simulink library "lib_IC_VSM"  (R2026a)
settings: Solver=VariableStepAuto
undefined symbols (not defined in the file): block_buses, block_DC_buses, block_DC_toM, block_idx, block_toM, buses_lf, DC, dparams, fb, fref, iC, inv2Hv, invL, iR, iTf, omegab, op_intconv_VSM
libraries: sl_discontinuities x1
(part 2 of 3)

== system lib_IC_VSM/intconv_VSM/VI/WOF_q ==
  note: 1) Add Subsystem or Model blocks as valid variant choices.
      | 2) You cannot connect blocks at this level. At simulation, connectivity is automatically
      | determined, based on the active variant and port name matching.
  In1 : Inport
  Active : Subsystem  VariantControl=use_Tf == 1
  Bypass : Subsystem  VariantControl=(default)
  Out1 : Outport

== system lib_IC_VSM/intconv_VSM/DC_ATM_Control/Int_kiw/Active ==
  In1 : Inport
  Impl : Integrator  InitialCondition=op_intconv_VSM.DC_ATM_Control_Int_kiw_Active_Impl
  Out1 : Outport
  wires:
  Impl/1 -> Out1/1
  In1/1 -> Impl/1

== system lib_IC_VSM/intconv_VSM/DC_ATM_Control/Int_kiw/Bypass ==
  In1 : Inport
  Out1 : Outport
  wires:
  In1/1 -> Out1/1

== system lib_IC_VSM/intconv_VSM/DC_ATM_Control/WOF_dc/Active ==
  In1 : Inport
  Impl : Subsystem
  Out1 : Outport
  wires:
  Impl/1(Out1) -> Out1/1
  In1/1 -> Impl/1(In1)

== system lib_IC_VSM/intconv_VSM/DC_ATM_Control/WOF_dc/Bypass ==
  In1 : Inport
  Out1 : Outport
  wires:
  In1/1 -> Out1/1

== system lib_IC_VSM/intconv_VSM/PC/LPF_P/Active ==
  In1 : Inport
  Impl : Subsystem
  Out1 : Outport
  wires:
  Impl/1(P_f) -> Out1/1
  In1/1 -> Impl/1(P)

== system lib_IC_VSM/intconv_VSM/PC/LPF_P/Bypass ==
  In1 : Inport
  Out1 : Outport
  wires:
  In1/1 -> Out1/1

== system lib_IC_VSM/intconv_VSM/PC/LPF_Q/Active ==
  In1 : Inport
  Impl : Subsystem
  Out1 : Outport
  wires:
  Impl/1(Q_f) -> Out1/1
  In1/1 -> Impl/1(Q)

== system lib_IC_VSM/intconv_VSM/PC/LPF_Q/Bypass ==
  In1 : Inport
  Out1 : Outport
  wires:
  In1/1 -> Out1/1

== system lib_IC_VSM/intconv_VSM/PC/Swing/Active ==
  Psp : Inport
  P_f : Inport  Port=2
  omegaref : Inport  Port=3
  Gain_Dv : Gain  Gain=Dv
  Gain_inv2Hv : Gain  Gain=inv2Hv
  Gain_invRv : Gain  Gain=1./Rv
  One_w : Constant  Value=ones(1, length(block_buses))  VectorParams1D=off
  Sum_acc : Sum  Inputs=+---
  Sum_dw_1 : Sum  Inputs=+-
  Sum_dw_ref : Sum  Inputs=+-
  omega_i : Integrator  InitialCondition=op_intconv_VSM.PC_omega_i
  y : Outport
  wires:
  Psp/1 -> Sum_acc/1
  P_f/1 -> Sum_acc/2
  omega_i/1 -> Sum_dw_ref/1, Sum_dw_1/1, y/1
  omegaref/1 -> Sum_dw_ref/2
  Sum_dw_ref/1 -> Gain_invRv/1
  Gain_invRv/1 -> Sum_acc/3
  One_w/1 -> Sum_dw_1/2
  Sum_dw_1/1 -> Gain_Dv/1
  Gain_Dv/1 -> Sum_acc/4
  Sum_acc/1 -> Gain_inv2Hv/1
  Gain_inv2Hv/1 -> omega_i/1

== system lib_IC_VSM/intconv_VSM/PC/Swing/Droop ==
  Psp : Inport
  P_f : Inport  Port=2
  omegaref : Inport  Port=3
  Gain_Rv : Gain  Gain=Rv
  Sum_P : Sum  Inputs=+-
  Sum_w : Sum
  y : Outport
  wires:
  Psp/1 -> Sum_P/1
  P_f/1 -> Sum_P/2
  Sum_P/1 -> Gain_Rv/1
  Gain_Rv/1 -> Sum_w/1
  omegaref/1 -> Sum_w/2
  Sum_w/1 -> y/1

== system lib_IC_VSM/intconv_VSM/VCC/dynamic/PIid ==
  ref : Inport
  y : Inport  Port=2
  Gain : Gain  Gain=Bint
  Gain1 : Gain  Gain=1./Tint
  Gain2 : Gain  Gain=Kint
  I : Integrator  InitialCondition=op_intconv_VSM.VCC_dynamic_PIid_I
  Sum : Sum  Inputs=++|
  Sum1 : Sum  Inputs=|+-
  Sum6 : Sum  Inputs=|+-
  Out1 : Outport
  wires:
  y/1 -> Sum1/2, Sum6/2
  ref/1 -> Gain/1, Sum6/1
  Gain/1 -> Sum1/1
  Sum/1 -> Gain2/1
  Sum1/1 -> Sum/1
  Sum6/1 -> Gain1/1
  Gain1/1 -> I/1
  I/1 -> Sum/2
  Gain2/1 -> Out1/1

== system lib_IC_VSM/intconv_VSM/VCC/dynamic/PIiq ==
  ref : Inport
  y : Inport  Port=2
  Gain : Gain  Gain=Bint
  Gain1 : Gain  Gain=1./Tint
  Gain2 : Gain  Gain=Kint
  I : Integrator  InitialCondition=op_intconv_VSM.VCC_dynamic_PIiq_I
  Sum : Sum  Inputs=++|
  Sum1 : Sum  Inputs=|+-
  Sum6 : Sum  Inputs=|+-
  Out1 : Outport
  wires:
  Gain2/1 -> Out1/1
  I/1 -> Sum/2
  Gain1/1 -> I/1
  Sum6/1 -> Gain1/1
  Sum1/1 -> Sum/1
  Sum/1 -> Gain2/1
  Gain/1 -> Sum1/1
  ref/1 -> Sum6/1, Gain/1
  y/1 -> Sum6/2, Sum1/2

== system lib_IC_VSM/intconv_VSM/VCC/dynamic/PIvd ==
  ref : Inport
  y : Inport  Port=2
  Gain : Gain  Gain=Bext
  Gain1 : Gain  Gain=1./Text
  Gain2 : Gain  Gain=Kext
  Integrator : Integrator  InitialCondition=op_intconv_VSM.VCC_dynamic_PIvd_Integrator
  Sum : Sum  Inputs=++|
  Sum1 : Sum  Inputs=|+-
  Sum6 : Sum  Inputs=|+-
  Out1 : Outport
  wires:
  y/1 -> Sum1/2, Sum6/2
  ref/1 -> Gain/1, Sum6/1
  Gain/1 -> Sum1/1
  Sum/1 -> Gain2/1
  Sum1/1 -> Sum/1
  Sum6/1 -> Gain1/1
  Gain1/1 -> Integrator/1
  Integrator/1 -> Sum/2
  Gain2/1 -> Out1/1

== system lib_IC_VSM/intconv_VSM/VCC/dynamic/PIvq ==
  ref : Inport
  y : Inport  Port=2
  Gain : Gain  Gain=Bext
  Gain1 : Gain  Gain=1./Text
  Gain2 : Gain  Gain=Kext
  Integrator : Integrator  InitialCondition=op_intconv_VSM.VCC_dynamic_PIvq_Integrator
  Sum : Sum  Inputs=++|
  Sum1 : Sum  Inputs=|+-
  Sum6 : Sum  Inputs=|+-
  Out1 : Outport
  wires:
  Gain2/1 -> Out1/1
  Integrator/1 -> Sum/2
  Gain1/1 -> Integrator/1
  Sum6/1 -> Gain1/1
  Sum1/1 -> Sum/1
  Sum/1 -> Gain2/1
  Gain/1 -> Sum1/1
  ref/1 -> Sum6/1, Gain/1
  y/1 -> Sum6/2, Sum1/2

== system lib_IC_VSM/intconv_VSM/VCC/dynamic/RC ==
  note: 1) Add Subsystem or Model blocks as valid variant choices.
      | 2) You cannot connect blocks at this level. At simulation, connectivity is automatically
      | determined, based on the active variant and port name matching.
  i_d_in : Inport
  i_d_out : Inport  Port=2
  i_q_in : Inport  Port=3
  i_q_out : Inport  Port=4
  omega : Inport  Port=5
  dynamic : Subsystem  VariantControl=rc_mode == 1  mask{v_d_0=1}
      mask prompts: v_d_0 "Initial condition for v_d"
  static : Subsystem  VariantControl=rc_mode == 2
  static omega : Subsystem  VariantControl=(default)
  vd : Outport
  vq : Outport  Port=2

== system lib_IC_VSM/intconv_VSM/VCC/dynamic/RL ==
  note: 1) Add Subsystem or Model blocks as valid variant choices.
      | 2) You cannot connect blocks at this level. At simulation, connectivity is automatically
      | determined, based on the active variant and port name matching.
  v_in_d : Inport
  v_out_d : Inport  Port=2
  v_in_q : Inport  Port=3
  v_out_q : Inport  Port=4
  dynamic : Subsystem  VariantControl=rl_mode == 1
      settings: PortSchema="{\"entries\":[{\"content\":{\"sides\":[{\"content\":{\"connectorIds\":[\"In1\"]},\"type\":\"ConnectorPlacement.EquallySpacedRectSide\",\"uuid\":\"63966e24-f9e7-4b2d-b456-7f4ea5e3f230\"},{\"content\":{\"connectorIds\":[\"In2\",\"In3\",\"In4\",\"Out1\",\"Out2\"],\"side\":\"RIGHT\"},\"type\":\"ConnectorPlacement.EquallySpacedRectSide\",\"uuid\":\"ded6ef04-52fd-47df-8e49-cf16b827098d\"},{\"content\":{\"connectorIds\":[],\"side\":\"TOP\"},\"type\":\"ConnectorPlacement.EquallySpacedRectSide\",\"uuid\":\"f940a985-fa23-4968-ad44-1d76d0e20c6a\"}]},\"type\":\"ConnectorPlacement.EquallySpacedConnector\",\"uuid\":\"20f61d3c-9af2-4982-98ea-af4910e61c9c\"}],\"packageUris\":[\"http://schema.mathworks.com/mf0/Connector/R2020b\"],\"version\":\"1.0\"}"
  static : Subsystem  VariantControl=rl_mode == 2
  static_omega : Subsystem  VariantControl=(default)
  id : Outport
  iq : Outport  Port=2

== system lib_IC_VSM/intconv_VSM/VCC/dynamic_VC/RC ==
  note: 1) Add Subsystem or Model blocks as valid variant choices.
      | 2) You cannot connect blocks at this level. At simulation, connectivity is automatically
      | determined, based on the active variant and port name matching.
  i_d_in : Inport
  i_d_out : Inport  Port=2
  i_q_in : Inport  Port=3
  i_q_out : Inport  Port=4
  omega : Inport  Port=5
  dynamic : Subsystem  VariantControl=rc_mode == 1  mask{v_d_0=1}
      mask prompts: v_d_0 "Initial condition for v_d"
  static : Subsystem  VariantControl=rc_mode == 2
  static omega : Subsystem  VariantControl=(default)
  v_d : Outport
  v_q : Outport  Port=2

== system lib_IC_VSM/intconv_VSM/VCC/dynamic_VC/Subsystem ==
  ref : Inport
  y : Inport  Port=2
  Gain : Gain  Gain=Bext
  Gain1 : Gain  Gain=1./Text
  Gain2 : Gain  Gain=Kext
  Integrator : Integrator  InitialCondition=op_intconv_VSM.VCC_dynamic_VC_Subsystem_Integrator
  Sum : Sum  Inputs=++|
  Sum1 : Sum  Inputs=|+-
  Sum6 : Sum  Inputs=|+-
  Out1 : Outport
  wires:
  y/1 -> Sum1/2, Sum6/2
  ref/1 -> Gain/1, Sum6/1
  Gain/1 -> Sum1/1
  Sum/1 -> Gain2/1
  Sum1/1 -> Sum/1
  Sum6/1 -> Gain1/1
  Gain1/1 -> Integrator/1
  Integrator/1 -> Sum/2
  Gain2/1 -> Out1/1

== system lib_IC_VSM/intconv_VSM/VCC/dynamic_VC/Subsystem1 ==
  ref : Inport
  y : Inport  Port=2
  Gain : Gain  Gain=Bext
  Gain1 : Gain  Gain=1./Text
  Gain2 : Gain  Gain=Kext
  Integrator : Integrator  InitialCondition=op_intconv_VSM.VCC_dynamic_VC_Subsystem1_Integrator
  Sum : Sum  Inputs=++|
  Sum1 : Sum  Inputs=|+-
  Sum6 : Sum  Inputs=|+-
  Out1 : Outport
  wires:
  Gain2/1 -> Out1/1
  Integrator/1 -> Sum/2
  Gain1/1 -> Integrator/1
  Sum6/1 -> Gain1/1
  Sum1/1 -> Sum/1
  Sum/1 -> Gain2/1
  Gain/1 -> Sum1/1
  ref/1 -> Sum6/1, Gain/1
  y/1 -> Sum6/2, Sum1/2

== system lib_IC_VSM/intconv_VSM/VCC/dynamic_limiting/PIid ==
  ref : Inport
  y : Inport  Port=2
  Gain : Gain  Gain=Bint
  Gain1 : Gain  Gain=1./Tint
  Gain2 : Gain  Gain=Kint
  I : Integrator  InitialCondition=op_intconv_VSM.VCC_dynamic_limiting_PIid_I
  Sum : Sum  Inputs=++|
  Sum1 : Sum  Inputs=|+-
  Sum6 : Sum  Inputs=|+-
  Out1 : Outport
  wires:
  y/1 -> Sum1/2, Sum6/2
  ref/1 -> Gain/1, Sum6/1
  Gain/1 -> Sum1/1
  Sum/1 -> Gain2/1
  Sum1/1 -> Sum/1
  Sum6/1 -> Gain1/1
  Gain1/1 -> I/1
  I/1 -> Sum/2
  Gain2/1 -> Out1/1

== system lib_IC_VSM/intconv_VSM/VCC/dynamic_limiting/PIiq ==
  ref : Inport
  y : Inport  Port=2
  Gain : Gain  Gain=Bint
  Gain1 : Gain  Gain=1./Tint
  Gain2 : Gain  Gain=Kint
  I : Integrator  InitialCondition=op_intconv_VSM.VCC_dynamic_limiting_PIiq_I
  Sum : Sum  Inputs=++|
  Sum1 : Sum  Inputs=|+-
  Sum6 : Sum  Inputs=|+-
  Out1 : Outport
  wires:
  Gain2/1 -> Out1/1
  I/1 -> Sum/2
  Gain1/1 -> I/1
  Sum6/1 -> Gain1/1
  Sum1/1 -> Sum/1
  Sum/1 -> Gain2/1
  Gain/1 -> Sum1/1
  ref/1 -> Sum6/1, Gain/1
  y/1 -> Sum6/2, Sum1/2

== system lib_IC_VSM/intconv_VSM/VCC/dynamic_limiting/PIvd ==
  ref : Inport
  y : Inport  Port=2
  anti_windup : Inport  Port=3
  Gain : Gain  Gain=Bext
  Gain1 : Gain  Gain=1./Text
  Gain2 : Gain  Gain=Kext
  I : Integrator  InitialCondition=op_intconv_VSM.VCC_dynamic_limiting_PIvd_I
  Product : Product
  Scope : Scope
      settings: ActiveDisplayYMinimum=-5E-5  ActiveDisplayYMaximum=0.00079  DataLoggingVariableName=ScopeData5
  Scope1 : Scope
      settings: ActiveDisplayYMinimum=-0.29497  ActiveDisplayYMaximum=2.2504  DataLoggingVariableName=ScopeData7
  Sum : Sum  Inputs=++|
  Sum1 : Sum  Inputs=|+-
  Sum6 : Sum  Inputs=|+-
  Out1 : Outport
  wires:
  y/1 -> Sum1/2, Sum6/2
  ref/1 -> Gain/1, Sum6/1
  Gain/1 -> Sum1/1
  Sum/1 -> Gain2/1
  Sum1/1 -> Sum/1
  Sum6/1 -> Scope1/1, Gain1/1
  Product/1 -> I/1
  I/1 -> Scope/1, Sum/2
  Gain2/1 -> Out1/1
  Gain1/1 -> Product/1
  anti_windup/1 -> Product/2

== system lib_IC_VSM/intconv_VSM/VCC/dynamic_limiting/PIvq ==
  ref : Inport
  y : Inport  Port=2
  anti_windup : Inport  Port=3
  Gain : Gain  Gain=Bext
  Gain1 : Gain  Gain=1./Text
  Gain2 : Gain  Gain=Kext
  I : Integrator  InitialCondition=op_intconv_VSM.VCC_dynamic_limiting_PIvq_I
  Product : Product
  Sum : Sum  Inputs=++|
  Sum1 : Sum  Inputs=|+-
  Sum6 : Sum  Inputs=|+-
  Out1 : Outport
  wires:
  Gain2/1 -> Out1/1
  I/1 -> Sum/2
  Product/1 -> I/1
  Sum6/1 -> Gain1/1
  Sum1/1 -> Sum/1
  Sum/1 -> Gain2/1
  Gain/1 -> Sum1/1
  ref/1 -> Sum6/1, Gain/1
  y/1 -> Sum6/2, Sum1/2
  Gain1/1 -> Product/1
  anti_windup/1 -> Product/2

== system lib_IC_VSM/intconv_VSM/VCC/dynamic_limiting/RC ==
  note: 1) Add Subsystem or Model blocks as valid variant choices.
      | 2) You cannot connect blocks at this level. At simulation, connectivity is automatically
      | determined, based on the active variant and port name matching.
  i_d_in : Inport
  i_d_out : Inport  Port=2
  i_q_in : Inport  Port=3
  i_q_out : Inport  Port=4
  omega : Inport  Port=5
  dynamic : Subsystem  VariantControl=rc_mode == 1
  static : Subsystem  VariantControl=rc_mode == 2
  static omega : Subsystem  VariantControl=(default)
  vd : Outport
  vq : Outport  Port=2

== system lib_IC_VSM/intconv_VSM/VCC/dynamic_limiting/RL ==
  note: 1) Add Subsystem or Model blocks as valid variant choices.
      | 2) You cannot connect blocks at this level. At simulation, connectivity is automatically
      | determined, based on the active variant and port name matching.
  v_in_d : Inport
  v_out_d : Inport  Port=2
  v_in_q : Inport  Port=3
  v_out_q : Inport  Port=4
  omega : Inport  Port=5
  dynamic : Subsystem  VariantControl=rl_mode == 1
      settings: PortSchema="{\"entries\":[{\"content\":{\"sides\":[{\"content\":{\"connectorIds\":[\"In1\"]},\"type\":\"ConnectorPlacement.EquallySpacedRectSide\",\"uuid\":\"63966e24-f9e7-4b2d-b456-7f4ea5e3f230\"},{\"content\":{\"connectorIds\":[\"In2\",\"In3\",\"In4\",\"In5\",\"Out1\",\"Out2\"],\"side\":\"RIGHT\"},\"type\":\"ConnectorPlacement.EquallySpacedRectSide\",\"uuid\":\"ded6ef04-52fd-47df-8e49-cf16b827098d\"},{\"content\":{\"side\":\"TOP\"},\"type\":\"ConnectorPlacement.EquallySpacedRectSide\",\"uuid\":\"f940a985-fa23-4968-ad44-1d76d0e20c6a\"}]},\"type\":\"ConnectorPlacement.EquallySpacedConnector\",\"uuid\":\"20f61d3c-9af2-4982-98ea-af4910e61c9c\"}],\"packageUris\":[\"http://schema.mathworks.com/mf0/Connector/R2020b\"],\"version\":\"1.0\"}"
  static : Subsystem  VariantControl=rl_mode == 2
  static_omega : Subsystem  VariantControl=(default)
  id : Outport
  iq : Outport  Port=2

== system lib_IC_VSM/intconv_VSM/VCC/dynamic_limiting/VI ==
  id : Inport
  iq : Inport  Port=2
  Gain : Gain  Gain=L
  Gain1 : Gain  Gain=R
  Gain2 : Gain  Gain=L
  Gain3 : Gain  Gain=R
  LPF_omega : Subsystem
  LPF_omega1 : Subsystem
  Sum : Sum  Inputs=-+|
  Sum1 : Sum  Inputs=|--
  WOF_d : Subsystem  Variant=on
  WOF_q : Subsystem  Variant=on
  vd : Outport
  vq : Outport  Port=2
  wires:
  WOF_q/1(Out1) -> Gain/1, Gain3/1
  iq/1 -> WOF_q/1(In1)
  WOF_d/1(Out1) -> Gain1/1, Gain2/1
  id/1 -> WOF_d/1(In1)
  Sum1/1 -> LPF_omega1/1(in)
  Sum/1 -> LPF_omega/1(in)
  Gain3/1 -> Sum1/2
  Gain1/1 -> Sum/1
  Gain2/1 -> Sum1/1
  Gain/1 -> Sum/2
  LPF_omega/1(out) -> vd/1
  LPF_omega1/1(out) -> vq/1

== system lib_IC_VSM/intconv_VSM/VCC/dynamic_limiting_P/PIid ==
  ref : Inport
  y : Inport  Port=2
  Gain : Gain  Gain=Bint
  Gain1 : Gain  Gain=1./Tint
  Gain2 : Gain  Gain=Kint
  I : Integrator  InitialCondition=op_intconv_VSM.VCC_dynamic_limiting_P_PIid_I
  Sum : Sum  Inputs=++|
  Sum1 : Sum  Inputs=|+-
  Sum6 : Sum  Inputs=|+-
  Out1 : Outport
  wires:
  y/1 -> Sum1/2, Sum6/2
  ref/1 -> Gain/1, Sum6/1
  Gain/1 -> Sum1/1
  Sum/1 -> Gain2/1
  Sum1/1 -> Sum/1
  Sum6/1 -> Gain1/1
  Gain1/1 -> I/1
  I/1 -> Sum/2
  Gain2/1 -> Out1/1

== system lib_IC_VSM/intconv_VSM/VCC/dynamic_limiting_P/PIiq ==
  ref : Inport
  y : Inport  Port=2
  Gain : Gain  Gain=Bint
  Gain1 : Gain  Gain=1./Tint
  Gain2 : Gain  Gain=Kint
  I : Integrator  InitialCondition=op_intconv_VSM.VCC_dynamic_limiting_P_PIiq_I
  Sum : Sum  Inputs=++|
  Sum1 : Sum  Inputs=|+-
  Sum6 : Sum  Inputs=|+-
  Out1 : Outport
  wires:
  Gain2/1 -> Out1/1
  I/1 -> Sum/2
  Gain1/1 -> I/1
  Sum6/1 -> Gain1/1
  Sum1/1 -> Sum/1
  Sum/1 -> Gain2/1
  Gain/1 -> Sum1/1
  ref/1 -> Sum6/1, Gain/1
  y/1 -> Sum6/2, Sum1/2

== system lib_IC_VSM/intconv_VSM/VCC/dynamic_limiting_P/PIvd ==
  ref : Inport
  y : Inport  Port=2
  awp : Inport  Port=3
  Gain : Gain  Gain=Bext
  Gain1 : Gain  Gain=1./Text
  Gain2 : Gain  Gain=Kext
  I : Integrator  InitialCondition=op_intconv_VSM.VCC_dynamic_limiting_P_PIvd_I
  Product : Product
  Sum : Sum  Inputs=++|
  Sum1 : Sum  Inputs=|+-
  Sum6 : Sum  Inputs=|+-
  Out1 : Outport
  wires:
  y/1 -> Sum1/2, Sum6/2
  ref/1 -> Gain/1, Sum6/1
  Gain/1 -> Sum1/1
  Sum/1 -> Gain2/1
  Sum1/1 -> Sum/1
  Sum6/1 -> Gain1/1
  Product/1 -> I/1
  Gain1/1 -> Product/1
  I/1 -> Sum/2
  awp/1 -> Product/2
  Gain2/1 -> Out1/1

== system lib_IC_VSM/intconv_VSM/VCC/dynamic_limiting_P/PIvq ==
  ref : Inport
  y : Inport  Port=2
  awp : Inport  Port=3
  Gain : Gain  Gain=Bext
  Gain1 : Gain  Gain=1./Text
  Gain2 : Gain  Gain=Kext
  I : Integrator  InitialCondition=op_intconv_VSM.VCC_dynamic_limiting_P_PIvq_I
  Product : Product
  Sum : Sum  Inputs=++|
  Sum1 : Sum  Inputs=|+-
  Sum6 : Sum  Inputs=|+-
  Out1 : Outport
  wires:
  I/1 -> Sum/2
  Sum6/1 -> Gain1/1
  Sum1/1 -> Sum/1
  Sum/1 -> Gain2/1
  Gain/1 -> Sum1/1
  ref/1 -> Sum6/1, Gain/1
  y/1 -> Sum6/2, Sum1/2
  Gain2/1 -> Out1/1
  Gain1/1 -> I/1, Product/1
  awp/1 -> Product/2

== system lib_IC_VSM/intconv_VSM/VCC/dynamic_limiting_P/RC ==
  note: 1) Add Subsystem or Model blocks as valid variant choices.
      | 2) You cannot connect blocks at this level. At simulation, connectivity is automatically
      | determined, based on the active variant and port name matching.
  i_d_in : Inport
  i_d_out : Inport  Port=2
  i_q_in : Inport  Port=3
  i_q_out : Inport  Port=4
  omega : Inport  Port=5
  dynamic : Subsystem  VariantControl=rc_mode == 1
  static : Subsystem  VariantControl=rc_mode == 2
  static omega : Subsystem  VariantControl=(default)
  vd : Outport
  vq : Outport  Port=2

== system lib_IC_VSM/intconv_VSM/VCC/dynamic_limiting_P/RL ==
  note: 1) Add Subsystem or Model blocks as valid variant choices.
      | 2) You cannot connect blocks at this level. At simulation, connectivity is automatically
      | determined, based on the active variant and port name matching.
  v_in_d : Inport
  v_out_d : Inport  Port=2
  v_in_q : Inport  Port=3
  v_out_q : Inport  Port=4
  omega : Inport  Port=5
  dynamic : Subsystem  VariantControl=rl_mode == 1
      settings: PortSchema="{\"entries\":[{\"content\":{\"sides\":[{\"content\":{\"connectorIds\":[\"In1\"]},\"type\":\"ConnectorPlacement.EquallySpacedRectSide\",\"uuid\":\"63966e24-f9e7-4b2d-b456-7f4ea5e3f230\"},{\"content\":{\"connectorIds\":[\"In2\",\"In3\",\"In4\",\"In5\",\"Out1\",\"Out2\"],\"side\":\"RIGHT\"},\"type\":\"ConnectorPlacement.EquallySpacedRectSide\",\"uuid\":\"ded6ef04-52fd-47df-8e49-cf16b827098d\"},{\"content\":{\"side\":\"TOP\"},\"type\":\"ConnectorPlacement.EquallySpacedRectSide\",\"uuid\":\"f940a985-fa23-4968-ad44-1d76d0e20c6a\"}]},\"type\":\"ConnectorPlacement.EquallySpacedConnector\",\"uuid\":\"20f61d3c-9af2-4982-98ea-af4910e61c9c\"}],\"packageUris\":[\"http://schema.mathworks.com/mf0/Connector/R2020b\"],\"version\":\"1.0\"}"
  static : Subsystem  VariantControl=rl_mode == 2
  static_omega : Subsystem  VariantControl=(default)
  id : Outport
  iq : Outport  Port=2

== system lib_IC_VSM/intconv_VSM/VCC/dynamic_limiting_P/Subsystem2 ==
  In1 : Inport
  In2 : Inport  Port=2
  imax : Inport  Port=3
  Complex to Magnitude-Angle1 : ComplexToMagnitudeAngle
  Complex to Real-Imag : ComplexToRealImag
  Constant1 : Constant  Value=0
  Magnitude-Angle to Complex : MagnitudeAngleToComplex
  Real-Imag to Complex2 : RealImagToComplex
  Relational Operator : RelationalOperator  Operator===  OutDataTypeStr=boolean  RndMeth=Simplest  InputSameDT=off
  Saturation Dynamic1 : sl_discontinuities/Saturation Dynamic  OutMin=[]  OutMax=[]  OutDataTypeStr=Inherit: Same as second input  OutDataType=fixdt(1, 16)  OutScaling=2^-10  DoSatur=off
  ref : Outport
  Out2 : Outport  Port=2
  awp : Outport  Port=3
  wires:
  Constant1/1 -> Saturation Dynamic1/3
  In1/1 -> Real-Imag to Complex2/1
  Complex to Magnitude-Angle1/2 -> Magnitude-Angle to Complex/2
  In2/1 -> Real-Imag to Complex2/2
  Saturation Dynamic1/1 -> Relational Operator/2, Magnitude-Angle to Complex/1
  Complex to Magnitude-Angle1/1 -> Relational Operator/1, Saturation Dynamic1/2
  imax/1 -> Saturation Dynamic1/1
  Magnitude-Angle to Complex/1 -> Complex to Real-Imag/1
  Real-Imag to Complex2/1 -> Complex to Magnitude-Angle1/1
  Complex to Real-Imag/1 -> ref/1
  Complex to Real-Imag/2 -> Out2/1
  Relational Operator/1 -> awp/1

== system lib_IC_VSM/intconv_VSM/VCC/dynamic_limiting_P/VI ==
  id : Inport
  iq : Inport  Port=2
  Gain : Gain  Gain=L
  Gain1 : Gain  Gain=R
  Gain2 : Gain  Gain=L
  Gain3 : Gain  Gain=R
  LPF_omega : Subsystem
  LPF_omega1 : Subsystem
  Sum : Sum  Inputs=-+|
  Sum1 : Sum  Inputs=|--
  WOF_d : Subsystem  Variant=on
  WOF_q : Subsystem  Variant=on
  vd : Outport
  vq : Outport  Port=2
  wires:
  WOF_q/1(Out1) -> Gain/1, Gain3/1
  iq/1 -> WOF_q/1(In1)
  WOF_d/1(Out1) -> Gain1/1, Gain2/1
  id/1 -> WOF_d/1(In1)
  Sum1/1 -> LPF_omega1/1(in)
  Sum/1 -> LPF_omega/1(in)
  Gain3/1 -> Sum1/2
  Gain1/1 -> Sum/1
  Gain2/1 -> Sum1/1
  Gain/1 -> Sum/2
  LPF_omega/1(out) -> vd/1
  LPF_omega1/1(out) -> vq/1

== system lib_IC_VSM/intconv_VSM/VI/WOF_d/Active ==
  In1 : Inport
  Impl : Subsystem
  Out1 : Outport
  wires:
  Impl/1(Out1) -> Out1/1
  In1/1 -> Impl/1(In1)

== system lib_IC_VSM/intconv_VSM/VI/WOF_d/Bypass ==
  In1 : Inport
  Out1 : Outport
  wires:
  In1/1 -> Out1/1

== system lib_IC_VSM/intconv_VSM/VI/WOF_q/Active ==
  In1 : Inport
  Impl : Subsystem
  Out1 : Outport
  wires:
  Impl/1(Out1) -> Out1/1
  In1/1 -> Impl/1(In1)

== system lib_IC_VSM/intconv_VSM/VI/WOF_q/Bypass ==
  In1 : Inport
  Out1 : Outport
  wires:
  In1/1 -> Out1/1

== system lib_IC_VSM/intconv_VSM/DC_ATM_Control/WOF_dc/Active/Impl ==
  In1 : Inport
  Gain : Gain  Gain=N_dc
  Gain1 : Gain  Gain=10
  I : Integrator  InitialConditionSource=external  InitialCondition=op_intconv_VSM.DC_ATM_Control_WOF_dc_Active_Impl_I
  Sum : Sum  Inputs=+-|
  Sum4 : Sum  Inputs=|+-
  Out1 : Outport
  wires:
  Gain/1 -> I/1
  Sum4/1 -> Gain/1
  In1/1 -> I/2, Sum/1, Sum4/1
  I/1 -> Sum/2, Sum4/2
  Sum/1 -> Gain1/1
  Gain1/1 -> Out1/1

== system lib_IC_VSM/intconv_VSM/PC/LPF_P/Active/Impl ==
  P : Inport
  Gain : Gain  Gain=iTf
  I : Integrator  InitialCondition=op_intconv_VSM.PC_LPF_P_Active_Impl_I
  Sum4 : Sum  Inputs=|+-
  P_f : Outport
  wires:
  I/1 -> Sum4/2, P_f/1
  P/1 -> Sum4/1
  Sum4/1 -> Gain/1
  Gain/1 -> I/1

== system lib_IC_VSM/intconv_VSM/PC/LPF_Q/Active/Impl ==
  Q : Inport
  Gain : Gain  Gain=iTf
  I : Integrator  InitialCondition=op_intconv_VSM.PC_LPF_Q_Active_Impl_I
  Sum4 : Sum  Inputs=|+-
  Q_f : Outport
  wires:
  Sum4/1 -> Gain/1
  I/1 -> Sum4/2, Q_f/1
  Q/1 -> Sum4/1
  Gain/1 -> I/1

== system lib_IC_VSM/intconv_VSM/VCC/dynamic/RC/dynamic ==
  omega : Inport
  i_d_in : Inport  Port=2
  i_d_out : Inport  Port=3
  i_q_in : Inport  Port=4
  i_q_out : Inport  Port=5
  Gain1 : Gain  Gain=iR
  Gain2 : Gain  Gain=iR
  Gain3 : Gain  Gain=C
  Gain4 : Gain  Gain=C
  Gain5 : Gain  Gain=iC.*omegab
  Gain6 : Gain  Gain=iC.*omegab
  Product : Product
  Product1 : Product
  Sum10 : Sum  Inputs=|-++
  Sum11 : Sum  Inputs=-+|
  Sum12 : Sum  Inputs=|+-
  Sum13 : Sum  Inputs=-+-|
  v_d : Integrator  InitialCondition=op_intconv_VSM.VCC_dynamic_RC_dynamic_v_d
  v_q : Integrator  InitialCondition=op_intconv_VSM.VCC_dynamic_RC_dynamic_v_q
  vd : Outport
  vq : Outport  Port=2
  wires:
  Sum10/1 -> Gain6/1
  Gain3/1 -> Product1/1
  v_q/1 -> vq/1, Gain2/1, Gain3/1  "vq"
  Product1/1 -> Sum10/3
  Gain4/1 -> Product/1
  Gain2/1 -> Sum13/3
  Product/1 -> Sum13/1
  Sum11/1 -> Sum10/2
  Gain6/1 -> v_d/1
  omega/1 -> Product/2, Product1/2  "omega"
  Sum13/1 -> Gain5/1
  Gain1/1 -> Sum10/1
  Gain5/1 -> v_q/1
  Sum12/1 -> Sum13/2
  v_d/1 -> Gain4/1, vd/1, Gain1/1  "vd"
  i_d_in/1 -> Sum11/2  "id1"
  i_d_out/1 -> Sum11/1  "id2"
  i_q_in/1 -> Sum12/1  "iq1"
  i_q_out/1 -> Sum12/2  "iq2"

== system lib_IC_VSM/intconv_VSM/VCC/dynamic/RC/static ==
  omega : Inport
  i_d_in : Inport  Port=2
  i_d_out : Inport  Port=3
  i_q_in : Inport  Port=4
  i_q_out : Inport  Port=5
  Constant : Constant  Value=iR.^2
  Constant1 : Constant
  Divide : Product  Inputs=*/
  Gain : Gain  Gain=C
  Gain1 : Gain  Gain=iR
  Gain2 : Gain  Gain=iR
  Product{,1..5} (6 alike) : Product
  Sum : Sum  Inputs=|++
  Sum1 : Sum  Inputs=|-+
  Sum2 : Sum  Inputs=|+-
  Sum3 : Sum  Inputs=|++
  Sum4 : Sum  Inputs=|-+
  vd : Outport
  vq : Outport  Port=2
  wires:
  Product5/1 -> Sum4/2
  Gain2/1 -> Product5/2
  Product4/1 -> Sum4/1
  Product2/1 -> Product3/1, Product4/2
  Product3/1 -> Sum3/2
  Product1/1 -> Sum3/1
  Divide/1 -> Product2/1, Gain1/1, Product5/1
  Gain1/1 -> Product1/2
  Sum2/1 -> Product3/2, Gain2/1  "iq"
  Sum1/1 -> Product4/1, Product1/1  "id"
  Constant1/1 -> Divide/1
  Product/1 -> Sum/2
  Gain/1 -> Product/1, Product/2, Product2/2
  Sum/1 -> Divide/2
  Constant/1 -> Sum/1
  Sum4/1 -> vq/1  "vq"
  Sum3/1 -> vd/1  "vd"
  omega/1 -> Gain/1  "omega"
  i_d_in/1 -> Sum1/2  "id1"
  i_q_in/1 -> Sum1/1  "id2"
  i_d_out/1 -> Sum2/1  "iq1"
  i_q_out/1 -> Sum2/2  "iq2"

== system lib_IC_VSM/intconv_VSM/VCC/dynamic/RC/static omega ==
  i_d_in : Inport
  i_d_out : Inport  Port=2
  i_q_in : Inport  Port=3
  i_q_out : Inport  Port=4
  Gain : Gain  Gain=1./(iR.^2+C.^2)
  Gain2 : Gain  Gain=1./(iR.^2+C.^2)
  Gain3 : Gain  Gain=iR
  Gain4 : Gain  Gain=C
  Gain5 : Gain  Gain=iR
  Gain6 : Gain  Gain=C
  Sum : Sum  Inputs=|++
  Sum1 : Sum  Inputs=|+-
  Sum2 : Sum  Inputs=|+-
  Sum4 : Sum  Inputs=|-+
  vd : Outport
  vq : Outport  Port=2
  wires:
  i_q_in/1 -> Sum2/1  "iq1"
  Sum1/1 -> Gain/1  "id"
  Sum2/1 -> Gain2/1  "iq"
  i_q_out/1 -> Sum2/2  "iq2"
  i_d_in/1 -> Sum1/1  "id"
  i_d_out/1 -> Sum1/2
  Gain/1 -> Gain4/1, Gain3/1
  Gain2/1 -> Gain6/1, Gain5/1
  Gain3/1 -> Sum/1
  Gain6/1 -> Sum/2
  Gain4/1 -> Sum4/1
  Gain5/1 -> Sum4/2
  Sum4/1 -> vq/1
  Sum/1 -> vd/1

== system lib_IC_VSM/intconv_VSM/VCC/dynamic/RL/dynamic ==
  v_in_d : Inport
  v_out_d : Inport  Port=2
  v_in_q : Inport  Port=3
  v_out_q : Inport  Port=4
  Gain1 : Gain  Gain=L
  Gain2 : Gain  Gain=R
  Gain3 : Gain  Gain=R
  Gain4 : Gain  Gain=L
  Gain5 : Gain  Gain=invL.*omegab
  Gain7 : Gain  Gain=invL.*omegab
  Product : Product
  Product1 : Product
  Sum4 : Sum  Inputs=+-|
  Sum5 : Sum  Inputs=|-+
  Sum6 : Sum  Inputs=|++
  Sum7 : Sum  Inputs=-+|
  Sum8 : Sum  Inputs=|+-
  Sum9 : Sum  Inputs=-+|
  i_d : Integrator  InitialCondition=op_intconv_VSM.VCC_dynamic_RL_dynamic_i_d
  i_q : Integrator  InitialCondition=op_intconv_VSM.VCC_dynamic_RL_dynamic_i_q
  id : Outport
  iq : Outport  Port=2
  wires:
  v_out_q/1 -> Sum9/1  "v_out_q"
  v_out_d/1 -> Sum7/1  "v_out_d"
  Sum9/1 -> Sum8/1
  Gain1/1 -> Product1/2
  i_q/1 -> iq/1, Gain4/1, Gain3/1  "iq"
  Gain7/1 -> i_q/1
  Sum5/1 -> Sum9/2
  Gain3/1 -> Sum5/1
  Sum7/1 -> Sum6/1
  Gain4/1 -> Product/1
  Product1/1 -> Sum8/2
  Sum4/1 -> Sum7/2
  Sum8/1 -> Gain7/1
  Product/1 -> Sum6/2
  Gain5/1 -> i_d/1
  [omega_ref] -> Product/2, Product1/1  "omega"
  Sum6/1 -> Gain5/1
  i_d/1 -> id/1, Gain1/1, Gain2/1  "id"
  Gain2/1 -> Sum4/2
  v_in_d/1 -> Sum4/1  "v_in_d"
  v_in_q/1 -> Sum5/2  "v_in_q"

== system lib_IC_VSM/intconv_VSM/VCC/dynamic/RL/static ==
  v_in_d : Inport
  v_out_d : Inport  Port=2
  v_in_q : Inport  Port=3
  v_out_q : Inport  Port=4
  Constant : Constant  Value=R.^2
  Constant1 : Constant
  Divide : Product  Inputs=*/
  Gain : Gain  Gain=L
  Gain1 : Gain  Gain=R
  Gain2 : Gain  Gain=R
  Product{,1..5} (6 alike) : Product
  Sum : Sum  Inputs=|++
  Sum1 : Sum  Inputs=|+-
  Sum2 : Sum  Inputs=|+-
  Sum3 : Sum  Inputs=|++
  Sum4 : Sum  Inputs=|-+
  id : Outport
  iq : Outport  Port=2
  wires:
  [omega_ref] -> Gain/1  "omega"
  v_in_d/1 -> Sum1/1  "v_in_d"
  v_out_q/1 -> Sum2/2  "v_out_q"
  Sum4/1 -> iq/1  "iq"
  Sum3/1 -> id/1  "id"
  Gain1/1 -> Product1/2
  Product2/1 -> Product4/2, Product3/1
  Product4/1 -> Sum4/1
  Divide/1 -> Gain2/1, Gain1/1, Product2/1
  Sum1/1 -> Product1/1, Product4/1  "vd"
  Product3/1 -> Sum3/2
  Constant1/1 -> Divide/1
  Gain/1 -> Product/2, Product/1, Product2/2
  Sum2/1 -> Product5/1, Product3/2  "vq"
  Constant/1 -> Sum/1
  Product5/1 -> Sum4/2
  Product1/1 -> Sum3/1
  Product/1 -> Sum/2
  Gain2/1 -> Product5/2
  Sum/1 -> Divide/2
  v_out_d/1 -> Sum1/2  "v_out_d"
  v_in_q/1 -> Sum2/1  "v_in_q"

== system lib_IC_VSM/intconv_VSM/VCC/dynamic/RL/static_omega ==
  v_in_d : Inport
  v_out_d : Inport  Port=2
  v_in_q : Inport  Port=3
  v_out_q : Inport  Port=4
  Gain : Gain  Gain=1./(R.^2+L.^2)
  Gain2 : Gain  Gain=1./(R.^2+L.^2)
  Gain3 : Gain  Gain=R
  Gain4 : Gain  Gain=L
  Gain5 : Gain  Gain=L
  Gain6 : Gain  Gain=R
  Sum : Sum  Inputs=|++
  Sum1 : Sum  Inputs=|+-
  Sum2 : Sum  Inputs=|+-
  Sum3 : Sum  Inputs=|-+
  id : Outport
  iq : Outport  Port=2
  wires:
  v_in_q/1 -> Sum2/1  "v_in_q"
  v_in_d/1 -> Sum1/1  "v_in_d"
  v_out_q/1 -> Sum2/2  "v_out_q"
  v_out_d/1 -> Sum1/2  "v_out_d"
  Sum1/1 -> Gain/1  "vd"
  Sum2/1 -> Gain2/1  "vq"
  Gain/1 -> Gain5/1, Gain3/1
  Gain3/1 -> Sum/1
  Gain4/1 -> Sum/2
  Gain2/1 -> Gain6/1, Gain4/1
  Sum/1 -> id/1
  Gain5/1 -> Sum3/1
  Sum3/1 -> iq/1
  Gain6/1 -> Sum3/2

== system lib_IC_VSM/intconv_VSM/VCC/dynamic_VC/RC/dynamic ==
  omega : Inport
  i_d_in : Inport  Port=2
  i_d_out : Inport  Port=3
  i_q_in : Inport  Port=4
  i_q_out : Inport  Port=5
  Gain1 : Gain  Gain=iR
  Gain2 : Gain  Gain=iR
  Gain3 : Gain  Gain=C
  Gain4 : Gain  Gain=C
  Gain5 : Gain  Gain=iC.*omegab
  Gain6 : Gain  Gain=iC.*omegab
  Product : Product
  Product1 : Product
  Sum10 : Sum  Inputs=|-++
  Sum11 : Sum  Inputs=-+|
  Sum12 : Sum  Inputs=|+-
  Sum13 : Sum  Inputs=-+-|
  vd : Integrator  InitialCondition=op_intconv_VSM.VCC_dynamic_VC_RC_dynamic_vd
  vq : Integrator  InitialCondition=op_intconv_VSM.VCC_dynamic_VC_RC_dynamic_vq
  v_d : Outport
  v_q : Outport  Port=2
  wires:
  Sum10/1 -> Gain6/1
  Gain3/1 -> Product1/1
  vq/1 -> v_q/1, Gain2/1, Gain3/1  "vq"
  Product1/1 -> Sum10/3
  Gain4/1 -> Product/1
  Gain2/1 -> Sum13/3
  Product/1 -> Sum13/1
  Sum11/1 -> Sum10/2
  Gain6/1 -> vd/1
  omega/1 -> Product/2, Product1/2  "omega"
  Sum13/1 -> Gain5/1
  Gain1/1 -> Sum10/1
  Gain5/1 -> vq/1
  Sum12/1 -> Sum13/2
  vd/1 -> Gain4/1, v_d/1, Gain1/1  "vd"
  i_d_in/1 -> Sum11/2  "id1"
  i_d_out/1 -> Sum11/1  "id2"
  i_q_in/1 -> Sum12/1  "iq1"
  i_q_out/1 -> Sum12/2  "iq2"

== system lib_IC_VSM/intconv_VSM/VCC/dynamic_VC/RC/static ==
  omega : Inport
  i_d_in : Inport  Port=2
  i_d_out : Inport  Port=3
  i_q_in : Inport  Port=4
  i_q_out : Inport  Port=5
  Constant : Constant  Value=iR.^2
  Constant1 : Constant
  Divide : Product  Inputs=*/
  Gain : Gain  Gain=C
  Gain1 : Gain  Gain=iR
  Gain2 : Gain  Gain=iR
  Product{,1..5} (6 alike) : Product
  Sum : Sum  Inputs=|++
  Sum1 : Sum  Inputs=|-+
  Sum2 : Sum  Inputs=|+-
  Sum3 : Sum  Inputs=|++
  Sum4 : Sum  Inputs=|-+
  v_d : Outport
  v_q : Outport  Port=2
  wires:
  Product5/1 -> Sum4/2
  Gain2/1 -> Product5/2
  Product4/1 -> Sum4/1
  Product2/1 -> Product3/1, Product4/2
  Product3/1 -> Sum3/2
  Product1/1 -> Sum3/1
  Divide/1 -> Product2/1, Gain1/1, Product5/1
  Gain1/1 -> Product1/2
  Sum2/1 -> Product3/2, Gain2/1  "iq"
  Sum1/1 -> Product4/1, Product1/1  "id"
  Constant1/1 -> Divide/1
  Product/1 -> Sum/2
  Gain/1 -> Product/1, Product/2, Product2/2
  Sum/1 -> Divide/2
  Constant/1 -> Sum/1
  Sum4/1 -> v_q/1  "vq"
  Sum3/1 -> v_d/1  "vd"
  omega/1 -> Gain/1  "omega"
  i_d_in/1 -> Sum1/2  "id1"
  i_d_out/1 -> Sum1/1  "id2"
  i_q_in/1 -> Sum2/1  "iq1"
  i_q_out/1 -> Sum2/2  "iq2"

== system lib_IC_VSM/intconv_VSM/VCC/dynamic_VC/RC/static omega ==
  i_d_in : Inport
  i_d_out : Inport  Port=2
  i_q_in : Inport  Port=3
  i_q_out : Inport  Port=4
  Gain : Gain  Gain=1./(iR.^2+C.^2)
  Gain2 : Gain  Gain=1./(iR.^2+C.^2)
  Gain3 : Gain  Gain=iR
  Gain4 : Gain  Gain=C
  Gain5 : Gain  Gain=iR
  Gain6 : Gain  Gain=C
  Sum : Sum  Inputs=|++
  Sum1 : Sum  Inputs=|+-
  Sum2 : Sum  Inputs=|+-
  Sum4 : Sum  Inputs=|-+
  v_d : Outport
  v_q : Outport  Port=2
  wires:
  i_q_in/1 -> Sum2/1  "iq1"
  Sum1/1 -> Gain/1  "id"
  Sum2/1 -> Gain2/1  "iq"
  i_q_out/1 -> Sum2/2  "iq2"
  i_d_in/1 -> Sum1/1  "id"
  i_d_out/1 -> Sum1/2
  Gain/1 -> Gain4/1, Gain3/1
  Gain2/1 -> Gain6/1, Gain5/1
  Gain3/1 -> Sum/1
  Gain6/1 -> Sum/2
  Gain4/1 -> Sum4/1
  Gain5/1 -> Sum4/2
  Sum4/1 -> v_q/1
  Sum/1 -> v_d/1

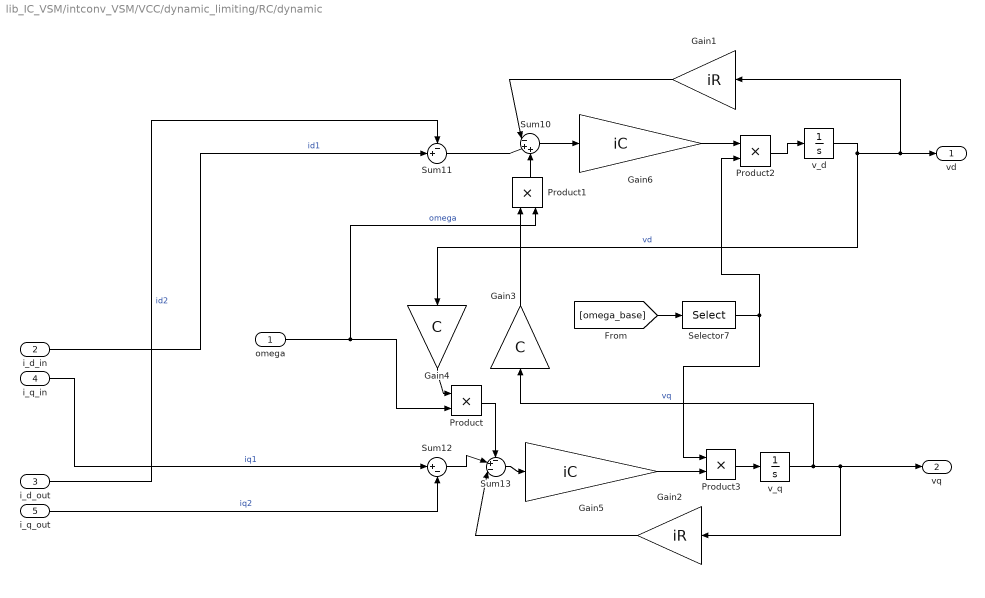
== system lib_IC_VSM/intconv_VSM/VCC/dynamic_limiting/RC/dynamic ==
  omega : Inport
  i_d_in : Inport  Port=2
  i_d_out : Inport  Port=3
  i_q_in : Inport  Port=4
  i_q_out : Inport  Port=5
  Gain1 : Gain  Gain=iR
  Gain2 : Gain  Gain=iR
  Gain3 : Gain  Gain=C
  Gain4 : Gain  Gain=C
  Gain5 : Gain  Gain=iC
  Gain6 : Gain  Gain=iC
  Product{,1..3} (4 alike) : Product
  Selector7 : Selector  InputPortWidth=length(fref.ref_units)  IndexOptions=Index vector (dialog)  Indices=block_fref  OutputSizes=1
  Sum10 : Sum  Inputs=|-++
  Sum11 : Sum  Inputs=-+|
  Sum12 : Sum  Inputs=|+-
  Sum13 : Sum  Inputs=-+-|
  v_d : Integrator  InitialCondition=op_intconv_VSM.VCC_dynamic_limiting_RC_dynamic_v_d
  v_q : Integrator  InitialCondition=op_intconv_VSM.VCC_dynamic_limiting_RC_dynamic_v_q
  vd : Outport
  vq : Outport  Port=2
  wires:
  Sum10/1 -> Gain6/1
  Gain3/1 -> Product1/1
  v_q/1 -> vq/1, Gain2/1, Gain3/1  "vq"
  Product1/1 -> Sum10/3
  Gain4/1 -> Product/1
  Gain2/1 -> Sum13/3
  Product/1 -> Sum13/1
  Sum11/1 -> Sum10/2
  omega/1 -> Product/2, Product1/2  "omega"
  Sum13/1 -> Gain5/1
  Gain1/1 -> Sum10/1
  Sum12/1 -> Sum13/2
  v_d/1 -> Gain4/1, vd/1, Gain1/1  "vd"
  i_d_in/1 -> Sum11/2  "id1"
  i_d_out/1 -> Sum11/1  "id2"
  i_q_in/1 -> Sum12/1  "iq1"
  i_q_out/1 -> Sum12/2  "iq2"
  [omega_base] -> Selector7/1
  Gain6/1 -> Product2/1
  Product2/1 -> v_d/1
  Selector7/1 -> Product2/2, Product3/1
  Product3/1 -> v_q/1
  Gain5/1 -> Product3/2

== system lib_IC_VSM/intconv_VSM/VCC/dynamic_limiting/RC/static ==
  omega : Inport
  i_d_in : Inport  Port=2
  i_d_out : Inport  Port=3
  i_q_in : Inport  Port=4
  i_q_out : Inport  Port=5
  Constant : Constant  Value=iR.^2
  Constant1 : Constant
  Divide : Product  Inputs=*/
  Gain : Gain  Gain=C
  Gain1 : Gain  Gain=iR
  Gain2 : Gain  Gain=iR
  Product{,1..5} (6 alike) : Product
  Sum : Sum  Inputs=|++
  Sum1 : Sum  Inputs=|-+
  Sum2 : Sum  Inputs=|+-
  Sum3 : Sum  Inputs=|++
  Sum4 : Sum  Inputs=|-+
  vd : Outport
  vq : Outport  Port=2
  wires:
  Product5/1 -> Sum4/2
  Gain2/1 -> Product5/2
  Product4/1 -> Sum4/1
  Product2/1 -> Product3/1, Product4/2
  Product3/1 -> Sum3/2
  Product1/1 -> Sum3/1
  Divide/1 -> Product2/1, Gain1/1, Product5/1
  Gain1/1 -> Product1/2
  Sum2/1 -> Product3/2, Gain2/1  "iq"
  Sum1/1 -> Product4/1, Product1/1  "id"
  Constant1/1 -> Divide/1
  Product/1 -> Sum/2
  Gain/1 -> Product/1, Product/2, Product2/2
  Sum/1 -> Divide/2
  Constant/1 -> Sum/1
  Sum4/1 -> vq/1  "vq"
  Sum3/1 -> vd/1  "vd"
  omega/1 -> Gain/1  "omega"
  i_d_in/1 -> Sum1/2  "id1"
  i_q_in/1 -> Sum1/1  "id2"
  i_d_out/1 -> Sum2/1  "iq1"
  i_q_out/1 -> Sum2/2  "iq2"

== system lib_IC_VSM/intconv_VSM/VCC/dynamic_limiting/RC/static omega ==
  i_d_in : Inport
  i_d_out : Inport  Port=2
  i_q_in : Inport  Port=3
  i_q_out : Inport  Port=4
  Gain : Gain  Gain=1./(iR.^2+C.^2)
  Gain2 : Gain  Gain=1./(iR.^2+C.^2)
  Gain3 : Gain  Gain=iR
  Gain4 : Gain  Gain=C
  Gain5 : Gain  Gain=iR
  Gain6 : Gain  Gain=C
  Sum : Sum  Inputs=|++
  Sum1 : Sum  Inputs=|+-
  Sum2 : Sum  Inputs=|+-
  Sum4 : Sum  Inputs=|-+
  vd : Outport
  vq : Outport  Port=2
  wires:
  i_q_in/1 -> Sum2/1  "iq1"
  Sum1/1 -> Gain/1  "id"
  Sum2/1 -> Gain2/1  "iq"
  i_q_out/1 -> Sum2/2  "iq2"
  i_d_in/1 -> Sum1/1  "id"
  i_d_out/1 -> Sum1/2
  Gain/1 -> Gain4/1, Gain3/1
  Gain2/1 -> Gain6/1, Gain5/1
  Gain3/1 -> Sum/1
  Gain6/1 -> Sum/2
  Gain4/1 -> Sum4/1
  Gain5/1 -> Sum4/2
  Sum4/1 -> vq/1
  Sum/1 -> vd/1

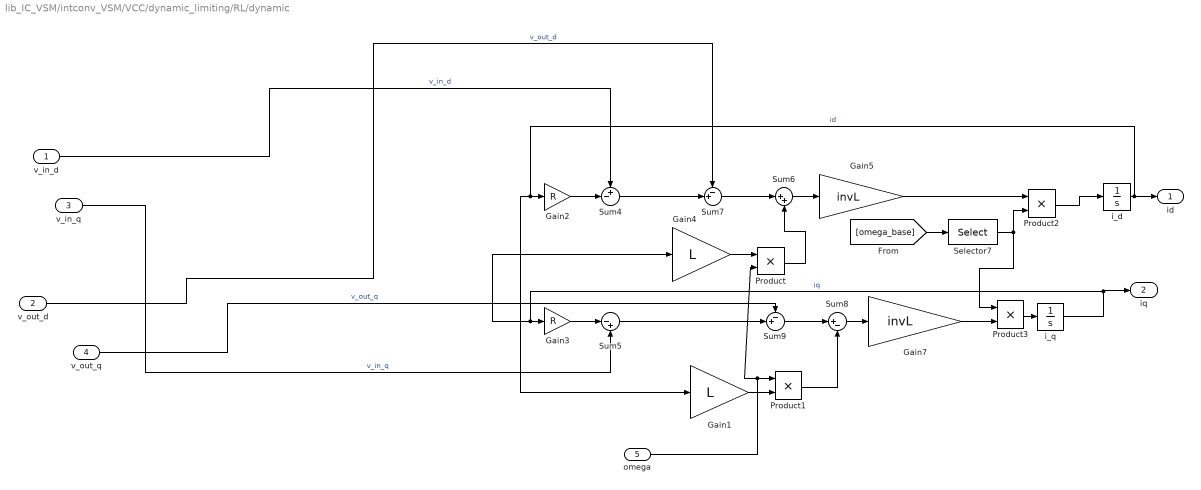
== system lib_IC_VSM/intconv_VSM/VCC/dynamic_limiting/RL/dynamic ==
  v_in_d : Inport
  v_out_d : Inport  Port=2
  v_in_q : Inport  Port=3
  v_out_q : Inport  Port=4
  omega : Inport  Port=5
  Gain1 : Gain  Gain=L
  Gain2 : Gain  Gain=R
  Gain3 : Gain  Gain=R
  Gain4 : Gain  Gain=L
  Gain5 : Gain  Gain=invL
  Gain7 : Gain  Gain=invL
  Product{,1..3} (4 alike) : Product
  Selector7 : Selector  InputPortWidth=length(fref.ref_units)  IndexOptions=Index vector (dialog)  Indices=block_fref  OutputSizes=1
  Sum4 : Sum  Inputs=+-|
  Sum5 : Sum  Inputs=|-+
  Sum6 : Sum  Inputs=|++
  Sum7 : Sum  Inputs=-+|
  Sum8 : Sum  Inputs=|+-
  Sum9 : Sum  Inputs=-+|
  i_d : Integrator  InitialCondition=op_intconv_VSM.VCC_dynamic_limiting_RL_dynamic_i_d
  i_q : Integrator  InitialCondition=op_intconv_VSM.VCC_dynamic_limiting_RL_dynamic_i_q
  id : Outport
  iq : Outport  Port=2
  wires:
  v_out_q/1 -> Sum9/1  "v_out_q"
  v_out_d/1 -> Sum7/1  "v_out_d"
  Sum9/1 -> Sum8/1
  Gain1/1 -> Product1/2
  i_q/1 -> iq/1, Gain4/1, Gain3/1  "iq"
  Gain7/1 -> Product3/2
  Sum5/1 -> Sum9/2
  Gain3/1 -> Sum5/1
  Sum7/1 -> Sum6/1
  Gain4/1 -> Product/1
  Product1/1 -> Sum8/2
  Sum4/1 -> Sum7/2
  Sum8/1 -> Gain7/1
  Product/1 -> Sum6/2
  Sum6/1 -> Gain5/1
  i_d/1 -> id/1, Gain1/1, Gain2/1  "id"
  Gain2/1 -> Sum4/2
  v_in_d/1 -> Sum4/1  "v_in_d"
  v_in_q/1 -> Sum5/2  "v_in_q"
  omega/1 -> Product/2, Product1/1
  Gain5/1 -> Product2/1
  Product2/1 -> i_d/1
  Selector7/1 -> Product2/2, Product3/1
  [omega_base] -> Selector7/1
  Product3/1 -> i_q/1

== system lib_IC_VSM/intconv_VSM/VCC/dynamic_limiting/RL/static ==
  v_in_d : Inport
  v_out_d : Inport  Port=2
  v_in_q : Inport  Port=3
  v_out_q : Inport  Port=4
  omega : Inport  Port=5
  Constant : Constant  Value=R.^2
  Constant1 : Constant
  Divide : Product  Inputs=*/
  Gain : Gain  Gain=L
  Gain1 : Gain  Gain=R
  Gain2 : Gain  Gain=R
  Product{,1..5} (6 alike) : Product
  Sum : Sum  Inputs=|++
  Sum1 : Sum  Inputs=|+-
  Sum2 : Sum  Inputs=|+-
  Sum3 : Sum  Inputs=|++
  Sum4 : Sum  Inputs=|-+
  id : Outport
  iq : Outport  Port=2
  wires:
  omega/1 -> Gain/1  "omega"
  v_in_d/1 -> Sum1/1  "v_in_d"
  v_out_q/1 -> Sum2/2  "v_out_q"
  Sum4/1 -> iq/1  "iq"
  Sum3/1 -> id/1  "id"
  Gain1/1 -> Product1/2
  Product2/1 -> Product4/2, Product3/1
  Product4/1 -> Sum4/1
  Divide/1 -> Gain2/1, Gain1/1, Product2/1
  Sum1/1 -> Product1/1, Product4/1  "vd"
  Product3/1 -> Sum3/2
  Constant1/1 -> Divide/1
  Gain/1 -> Product/2, Product/1, Product2/2
  Sum2/1 -> Product5/1, Product3/2  "vq"
  Constant/1 -> Sum/1
  Product5/1 -> Sum4/2
  Product1/1 -> Sum3/1
  Product/1 -> Sum/2
  Gain2/1 -> Product5/2
  Sum/1 -> Divide/2
  v_out_d/1 -> Sum1/2  "v_out_d"
  v_in_q/1 -> Sum2/1  "v_in_q"

== system lib_IC_VSM/intconv_VSM/VCC/dynamic_limiting/RL/static_omega ==
  v_in_d : Inport
  v_out_d : Inport  Port=2
  v_in_q : Inport  Port=3
  v_out_q : Inport  Port=4
  Gain : Gain  Gain=1./(R.^2+L.^2)
  Gain2 : Gain  Gain=1./(R.^2+L.^2)
  Gain3 : Gain  Gain=R
  Gain4 : Gain  Gain=L
  Gain5 : Gain  Gain=L
  Gain6 : Gain  Gain=R
  Sum : Sum  Inputs=|++
  Sum1 : Sum  Inputs=|+-
  Sum2 : Sum  Inputs=|+-
  Sum3 : Sum  Inputs=|-+
  id : Outport
  iq : Outport  Port=2
  wires:
  v_in_q/1 -> Sum2/1  "v_in_q"
  v_in_d/1 -> Sum1/1  "v_in_d"
  v_out_q/1 -> Sum2/2  "v_out_q"
  v_out_d/1 -> Sum1/2  "v_out_d"
  Sum1/1 -> Gain/1  "vd"
  Sum2/1 -> Gain2/1  "vq"
  Gain/1 -> Gain5/1, Gain3/1
  Gain3/1 -> Sum/1
  Gain4/1 -> Sum/2
  Gain2/1 -> Gain6/1, Gain4/1
  Sum/1 -> id/1
  Gain5/1 -> Sum3/1
  Sum3/1 -> iq/1
  Gain6/1 -> Sum3/2

== system lib_IC_VSM/intconv_VSM/VCC/dynamic_limiting/VI/LPF_omega ==
  in : Inport
  Gain : Gain  Gain=10
  I : Integrator  InitialCondition=op_intconv_VSM.VCC_dynamic_limiting_VI_LPF_omega_I
  Sum4 : Sum  Inputs=|+-
  out : Outport
  wires:
  Gain/1 -> I/1
  Sum4/1 -> Gain/1
  in/1 -> Sum4/1
  I/1 -> Sum4/2, out/1

== system lib_IC_VSM/intconv_VSM/VCC/dynamic_limiting/VI/LPF_omega1 ==
  in : Inport
  Gain : Gain  Gain=10
  I : Integrator  InitialCondition=op_intconv_VSM.VCC_dynamic_limiting_VI_LPF_omega1_I
  Sum4 : Sum  Inputs=|+-
  out : Outport
  wires:
  I/1 -> out/1, Sum4/2
  in/1 -> Sum4/1
  Sum4/1 -> Gain/1
  Gain/1 -> I/1

== system lib_IC_VSM/intconv_VSM/VCC/dynamic_limiting/VI/WOF_d ==
  note: 1) Add Subsystem or Model blocks as valid variant choices.
      | 2) You cannot connect blocks at this level. At simulation, connectivity is automatically
      | determined, based on the active variant and port name matching.
  In1 : Inport
  Active : Subsystem  VariantControl=use_Tf == 1
  Bypass : Subsystem  VariantControl=(default)
  Out1 : Outport

== system lib_IC_VSM/intconv_VSM/VCC/dynamic_limiting/VI/WOF_q ==
  note: 1) Add Subsystem or Model blocks as valid variant choices.
      | 2) You cannot connect blocks at this level. At simulation, connectivity is automatically
      | determined, based on the active variant and port name matching.
  In1 : Inport
  Active : Subsystem  VariantControl=use_Tf == 1
  Bypass : Subsystem  VariantControl=(default)
  Out1 : Outport

== system lib_IC_VSM/intconv_VSM/VCC/dynamic_limiting_P/RC/dynamic ==
  omega : Inport
  i_d_in : Inport  Port=2
  i_d_out : Inport  Port=3
  i_q_in : Inport  Port=4
  i_q_out : Inport  Port=5
  Gain1 : Gain  Gain=iR
  Gain2 : Gain  Gain=iR
  Gain3 : Gain  Gain=C
  Gain4 : Gain  Gain=C
  Gain5 : Gain  Gain=iC
  Gain6 : Gain  Gain=iC
  Product{,1..3} (4 alike) : Product
  Selector7 : Selector  InputPortWidth=length(fref.ref_units)  IndexOptions=Index vector (dialog)  Indices=block_fref  OutputSizes=1
  Sum10 : Sum  Inputs=|-++
  Sum11 : Sum  Inputs=-+|
  Sum12 : Sum  Inputs=|+-
  Sum13 : Sum  Inputs=-+-|
  v_d : Integrator  InitialCondition=op_intconv_VSM.VCC_dynamic_limiting_P_RC_dynamic_v_d
  v_q : Integrator  InitialCondition=op_intconv_VSM.VCC_dynamic_limiting_P_RC_dynamic_v_q
  vd : Outport
  vq : Outport  Port=2
  wires:
  Sum10/1 -> Gain6/1
  Gain3/1 -> Product1/1
  v_q/1 -> vq/1, Gain2/1, Gain3/1  "vq"
  Product1/1 -> Sum10/3
  Gain4/1 -> Product/1
  Gain2/1 -> Sum13/3
  Product/1 -> Sum13/1
  Sum11/1 -> Sum10/2
  omega/1 -> Product/2, Product1/2  "omega"
  Sum13/1 -> Gain5/1
  Gain1/1 -> Sum10/1
  Sum12/1 -> Sum13/2
  v_d/1 -> Gain4/1, vd/1, Gain1/1  "vd"
  i_d_in/1 -> Sum11/2  "id1"
  i_d_out/1 -> Sum11/1  "id2"
  i_q_in/1 -> Sum12/1  "iq1"
  i_q_out/1 -> Sum12/2  "iq2"
  [omega_base] -> Selector7/1
  Gain6/1 -> Product2/1
  Product2/1 -> v_d/1
  Selector7/1 -> Product2/2, Product3/1
  Product3/1 -> v_q/1
  Gain5/1 -> Product3/2

== system lib_IC_VSM/intconv_VSM/VCC/dynamic_limiting_P/RC/static ==
  omega : Inport
  i_d_in : Inport  Port=2
  i_d_out : Inport  Port=3
  i_q_in : Inport  Port=4
  i_q_out : Inport  Port=5
  Constant : Constant  Value=iR.^2
  Constant1 : Constant
  Divide : Product  Inputs=*/
  Gain : Gain  Gain=C
  Gain1 : Gain  Gain=iR
  Gain2 : Gain  Gain=iR
  Product{,1..5} (6 alike) : Product
  Sum : Sum  Inputs=|++
  Sum1 : Sum  Inputs=|-+
  Sum2 : Sum  Inputs=|+-
  Sum3 : Sum  Inputs=|++
  Sum4 : Sum  Inputs=|-+
  vd : Outport
  vq : Outport  Port=2
  wires:
  Product5/1 -> Sum4/2
  Gain2/1 -> Product5/2
  Product4/1 -> Sum4/1
  Product2/1 -> Product3/1, Product4/2
  Product3/1 -> Sum3/2
  Product1/1 -> Sum3/1
  Divide/1 -> Product2/1, Gain1/1, Product5/1
  Gain1/1 -> Product1/2
  Sum2/1 -> Product3/2, Gain2/1  "iq"
  Sum1/1 -> Product4/1, Product1/1  "id"
  Constant1/1 -> Divide/1
  Product/1 -> Sum/2
  Gain/1 -> Product/1, Product/2, Product2/2
  Sum/1 -> Divide/2
  Constant/1 -> Sum/1
  Sum4/1 -> vq/1  "vq"
  Sum3/1 -> vd/1  "vd"
  omega/1 -> Gain/1  "omega"
  i_d_in/1 -> Sum1/2  "id1"
  i_q_in/1 -> Sum1/1  "id2"
  i_d_out/1 -> Sum2/1  "iq1"
  i_q_out/1 -> Sum2/2  "iq2"

== system lib_IC_VSM/intconv_VSM/VCC/dynamic_limiting_P/RC/static omega ==
  i_d_in : Inport
  i_d_out : Inport  Port=2
  i_q_in : Inport  Port=3
  i_q_out : Inport  Port=4
  Gain : Gain  Gain=1./(iR.^2+C.^2)
  Gain2 : Gain  Gain=1./(iR.^2+C.^2)
  Gain3 : Gain  Gain=iR
  Gain4 : Gain  Gain=C
  Gain5 : Gain  Gain=iR
  Gain6 : Gain  Gain=C
  Sum : Sum  Inputs=|++
  Sum1 : Sum  Inputs=|+-
  Sum2 : Sum  Inputs=|+-
  Sum4 : Sum  Inputs=|-+
  vd : Outport
  vq : Outport  Port=2
  wires:
  i_q_in/1 -> Sum2/1  "iq1"
  Sum1/1 -> Gain/1  "id"
  Sum2/1 -> Gain2/1  "iq"
  i_q_out/1 -> Sum2/2  "iq2"
  i_d_in/1 -> Sum1/1  "id"
  i_d_out/1 -> Sum1/2
  Gain/1 -> Gain4/1, Gain3/1
  Gain2/1 -> Gain6/1, Gain5/1
  Gain3/1 -> Sum/1
  Gain6/1 -> Sum/2
  Gain4/1 -> Sum4/1
  Gain5/1 -> Sum4/2
  Sum4/1 -> vq/1
  Sum/1 -> vd/1

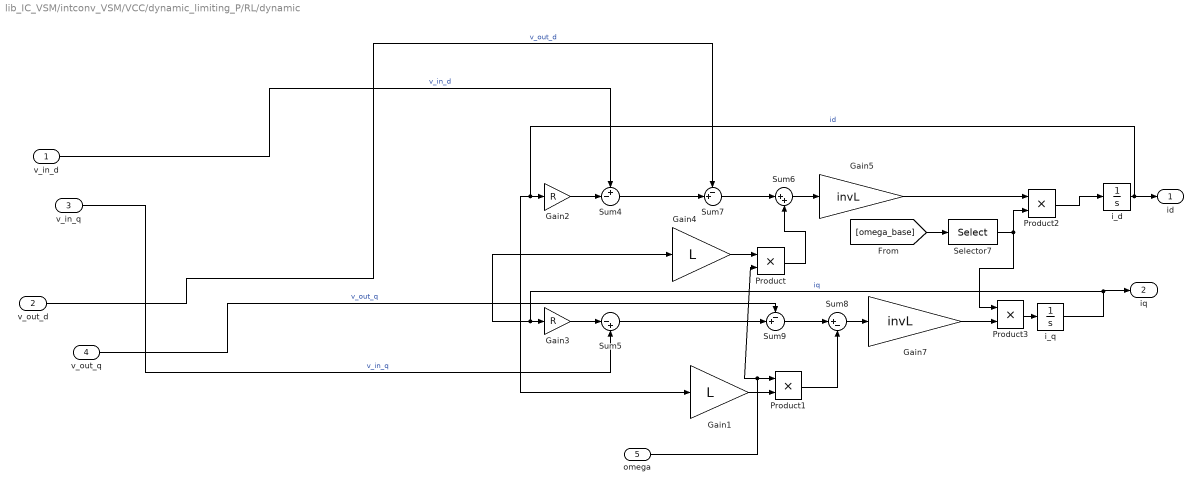
== system lib_IC_VSM/intconv_VSM/VCC/dynamic_limiting_P/RL/dynamic ==
  v_in_d : Inport
  v_out_d : Inport  Port=2
  v_in_q : Inport  Port=3
  v_out_q : Inport  Port=4
  omega : Inport  Port=5
  Gain1 : Gain  Gain=L
  Gain2 : Gain  Gain=R
  Gain3 : Gain  Gain=R
  Gain4 : Gain  Gain=L
  Gain5 : Gain  Gain=invL
  Gain7 : Gain  Gain=invL
  Product{,1..3} (4 alike) : Product
  Selector7 : Selector  InputPortWidth=length(fref.ref_units)  IndexOptions=Index vector (dialog)  Indices=block_fref  OutputSizes=1
  Sum4 : Sum  Inputs=+-|
  Sum5 : Sum  Inputs=|-+
  Sum6 : Sum  Inputs=|++
  Sum7 : Sum  Inputs=-+|
  Sum8 : Sum  Inputs=|+-
  Sum9 : Sum  Inputs=-+|
  i_d : Integrator  InitialCondition=op_intconv_VSM.VCC_dynamic_limiting_P_RL_dynamic_i_d
  i_q : Integrator  InitialCondition=op_intconv_VSM.VCC_dynamic_limiting_P_RL_dynamic_i_q
  id : Outport
  iq : Outport  Port=2
  wires:
  v_out_q/1 -> Sum9/1  "v_out_q"
  v_out_d/1 -> Sum7/1  "v_out_d"
  Sum9/1 -> Sum8/1
  Gain1/1 -> Product1/2
  i_q/1 -> iq/1, Gain4/1, Gain3/1  "iq"
  Gain7/1 -> Product3/2
  Sum5/1 -> Sum9/2
  Gain3/1 -> Sum5/1
  Sum7/1 -> Sum6/1
  Gain4/1 -> Product/1
  Product1/1 -> Sum8/2
  Sum4/1 -> Sum7/2
  Sum8/1 -> Gain7/1
  Product/1 -> Sum6/2
  Sum6/1 -> Gain5/1
  i_d/1 -> id/1, Gain1/1, Gain2/1  "id"
  Gain2/1 -> Sum4/2
  v_in_d/1 -> Sum4/1  "v_in_d"
  v_in_q/1 -> Sum5/2  "v_in_q"
  omega/1 -> Product/2, Product1/1
  Gain5/1 -> Product2/1
  Product2/1 -> i_d/1
  Selector7/1 -> Product2/2, Product3/1
  [omega_base] -> Selector7/1
  Product3/1 -> i_q/1

== system lib_IC_VSM/intconv_VSM/VCC/dynamic_limiting_P/RL/static ==
  v_in_d : Inport
  v_out_d : Inport  Port=2
  v_in_q : Inport  Port=3
  v_out_q : Inport  Port=4
  omega : Inport  Port=5
  Constant : Constant  Value=R.^2
  Constant1 : Constant
  Divide : Product  Inputs=*/
  Gain : Gain  Gain=L
  Gain1 : Gain  Gain=R
  Gain2 : Gain  Gain=R
  Product{,1..5} (6 alike) : Product
  Sum : Sum  Inputs=|++
  Sum1 : Sum  Inputs=|+-
  Sum2 : Sum  Inputs=|+-
  Sum3 : Sum  Inputs=|++
  Sum4 : Sum  Inputs=|-+
  id : Outport
  iq : Outport  Port=2
  wires:
  omega/1 -> Gain/1  "omega"
  v_in_d/1 -> Sum1/1  "v_in_d"
  v_out_q/1 -> Sum2/2  "v_out_q"
  Sum4/1 -> iq/1  "iq"
  Sum3/1 -> id/1  "id"
  Gain1/1 -> Product1/2
  Product2/1 -> Product4/2, Product3/1
  Product4/1 -> Sum4/1
  Divide/1 -> Gain2/1, Gain1/1, Product2/1
  Sum1/1 -> Product1/1, Product4/1  "vd"
  Product3/1 -> Sum3/2
  Constant1/1 -> Divide/1
  Gain/1 -> Product/2, Product/1, Product2/2
  Sum2/1 -> Product5/1, Product3/2  "vq"
  Constant/1 -> Sum/1
  Product5/1 -> Sum4/2
  Product1/1 -> Sum3/1
  Product/1 -> Sum/2
  Gain2/1 -> Product5/2
  Sum/1 -> Divide/2
  v_out_d/1 -> Sum1/2  "v_out_d"
  v_in_q/1 -> Sum2/1  "v_in_q"

== system lib_IC_VSM/intconv_VSM/VCC/dynamic_limiting_P/RL/static_omega ==
  v_in_d : Inport
  v_out_d : Inport  Port=2
  v_in_q : Inport  Port=3
  v_out_q : Inport  Port=4
  Gain : Gain  Gain=1./(R.^2+L.^2)
  Gain2 : Gain  Gain=1./(R.^2+L.^2)
  Gain3 : Gain  Gain=R
  Gain4 : Gain  Gain=L
  Gain5 : Gain  Gain=L
  Gain6 : Gain  Gain=R
  Sum : Sum  Inputs=|++
  Sum1 : Sum  Inputs=|+-
  Sum2 : Sum  Inputs=|+-
  Sum3 : Sum  Inputs=|-+
  id : Outport
  iq : Outport  Port=2
  wires:
  v_in_q/1 -> Sum2/1  "v_in_q"
  v_in_d/1 -> Sum1/1  "v_in_d"
  v_out_q/1 -> Sum2/2  "v_out_q"
  v_out_d/1 -> Sum1/2  "v_out_d"
  Sum1/1 -> Gain/1  "vd"
  Sum2/1 -> Gain2/1  "vq"
  Gain/1 -> Gain5/1, Gain3/1
  Gain3/1 -> Sum/1
  Gain4/1 -> Sum/2
  Gain2/1 -> Gain6/1, Gain4/1
  Sum/1 -> id/1
  Gain5/1 -> Sum3/1
  Sum3/1 -> iq/1
  Gain6/1 -> Sum3/2

== system lib_IC_VSM/intconv_VSM/VCC/dynamic_limiting_P/VI/LPF_omega ==
  in : Inport
  Gain : Gain  Gain=10
  I : Integrator  InitialCondition=op_intconv_VSM.VCC_dynamic_limiting_P_VI_LPF_omega_I
  Sum4 : Sum  Inputs=|+-
  out : Outport
  wires:
  Gain/1 -> I/1
  Sum4/1 -> Gain/1
  in/1 -> Sum4/1
  I/1 -> Sum4/2, out/1

== system lib_IC_VSM/intconv_VSM/VCC/dynamic_limiting_P/VI/LPF_omega1 ==
  in : Inport
  Gain : Gain  Gain=10
  I : Integrator  InitialCondition=op_intconv_VSM.VCC_dynamic_limiting_P_VI_LPF_omega1_I
  Sum4 : Sum  Inputs=|+-
  out : Outport
  wires:
  I/1 -> out/1, Sum4/2
  in/1 -> Sum4/1
  Sum4/1 -> Gain/1
  Gain/1 -> I/1

== system lib_IC_VSM/intconv_VSM/VCC/dynamic_limiting_P/VI/WOF_d ==
  note: 1) Add Subsystem or Model blocks as valid variant choices.
      | 2) You cannot connect blocks at this level. At simulation, connectivity is automatically
      | determined, based on the active variant and port name matching.
  In1 : Inport
  Active : Subsystem  VariantControl=use_Tf == 1
  Bypass : Subsystem  VariantControl=(default)
  Out1 : Outport

== system lib_IC_VSM/intconv_VSM/VCC/dynamic_limiting_P/VI/WOF_q ==
  note: 1) Add Subsystem or Model blocks as valid variant choices.
      | 2) You cannot connect blocks at this level. At simulation, connectivity is automatically
      | determined, based on the active variant and port name matching.
  In1 : Inport
  Active : Subsystem  VariantControl=use_Tf == 1
  Bypass : Subsystem  VariantControl=(default)
  Out1 : Outport

== system lib_IC_VSM/intconv_VSM/VI/WOF_d/Active/Impl ==
  In1 : Inport
  Gain : Gain  Gain=iTf
  I : Integrator  InitialConditionSource=external  InitialCondition=op_intconv_VSM.VI_WOF_d_Active_Impl_I
  Sum : Sum  Inputs=+-|
  Sum4 : Sum  Inputs=|+-
  Out1 : Outport
  wires:
  Gain/1 -> I/1
  Sum4/1 -> Gain/1
  In1/1 -> I/2, Sum/1, Sum4/1
  I/1 -> Sum/2, Sum4/2
  Sum/1 -> Out1/1

== system lib_IC_VSM/intconv_VSM/VI/WOF_q/Active/Impl ==
  In1 : Inport
  Gain : Gain  Gain=iTf
  I : Integrator  InitialConditionSource=external  InitialCondition=op_intconv_VSM.VI_WOF_q_Active_Impl_I
  Sum : Sum  Inputs=+-|
  Sum4 : Sum  Inputs=|+-
  Out1 : Outport
  wires:
  Gain/1 -> I/1
  Sum4/1 -> Gain/1
  In1/1 -> I/2, Sum/1, Sum4/1
  I/1 -> Sum/2, Sum4/2
  Sum/1 -> Out1/1

== system lib_IC_VSM/intconv_VSM/VCC/dynamic_limiting/VI/WOF_d/Active ==
  In1 : Inport
  Impl : Subsystem
  Out1 : Outport
  wires:
  Impl/1(Out1) -> Out1/1
  In1/1 -> Impl/1(In1)

== system lib_IC_VSM/intconv_VSM/VCC/dynamic_limiting/VI/WOF_d/Bypass ==
  In1 : Inport
  Out1 : Outport
  wires:
  In1/1 -> Out1/1

== system lib_IC_VSM/intconv_VSM/VCC/dynamic_limiting/VI/WOF_q/Active ==
  In1 : Inport
  Impl : Subsystem
  Out1 : Outport
  wires:
  Impl/1(Out1) -> Out1/1
  In1/1 -> Impl/1(In1)
